simulink model "XROBO02_reference"  (R2025a)
settings: Solver=ode15s  StartTime=0  StopTime=8  MaxStep=0.002  RelTol=1e-3  AbsTol=1e-3
undefined symbols (not defined in the file): cube_l, disturbance_start, disturbance_torque_nm, F1, F2, left_target_rad, move_duration, right_target_rad, shared_payload_mass, torque_limit_scale, X, Y, Z
libraries: sm_lib x210, nesl_utility x45
(part 1 of 5)
CloseFcn:
  | try,close(h1_sm_abbYuMi_trajectory),end
  | clear h1_sm_abbYuMi_2_trajectory
  | try,close(h2_sm_abbYuMi_trajectory),end
  | clear h2_sm_abbYuMi_2_trajectory
  | try,close(h3_sm_abbYuMi_trajectory),end
  | clear h3_sm_abbYuMi_2_trajectory
  | try,close(h4_sm_abbYuMi_trajectory),end
  | clear h4_sm_abbYuMi_trajectory
  | 
  | 
  | clear simlog_sm_abbYuMi_trajectory
  | clear logsout_sm_abbYuMi_trajectory
Description:
  | Dual Arm Robot Trajectory Testing
  | Copyright 2021-2025 The MathWorks, Inc.
settings Model: Creator=smiller  LastModifiedBy=SimuVerity Contributors
settings SolverCC: AutoScaleAbsTol=off
settings DataIOCC: MaxDataPoints=10000  SignalLoggingName=logsout_sm_abbYuMi_trajectory
settings OptimizationCC: ReuseModelBlockBuffer=off
settings DebuggingCC: UnconnectedInputMsg=warning  UnconnectedOutputMsg=warning  UnconnectedLineMsg=warning
settings ModelReferenceCC: EnableRefExpFcnMdlSchedulingChecks=on
settings RTWCC: GPUComputeCapability=3.5  DLArmComputeVersion=19.05
settings SimscapeCC: SimscapeLogSimulationStatistics=on  SimscapeLogName=simlog_sm_abbYuMi_trajectory  SimscapeLogDataHistory=10000.0
settings ExplorerConfigSet: InternalSimMechanicsExplorerSettings="<ExplorerConfiguration><canonicalview>default</canonicalview><AnimationSetting><BasePlaybackSpeed>1.0</BasePlaybackSpeed><PlaybackSpeedFactor>1.0</PlaybackSpeedFactor></AnimationSetting><TilePanel><TileInfo><Tiles Columns=\"3\" Count=\"4\" Rows=\"2\"><Column Weight=\"0.6174\"/><Column Weight=\"0.1908\"/><Column Weight=\"0.1918\"/><Row Weight=\"0.4992\"/><Row Weight=\"0.5008\"/><Tile Height=\"2\" Width=\"1\" X=\"0\" Y=\"0\"/><Tile Height=\"1\" Width=\"1\" X=\"1\" Y=\"0\"/><Tile Height=\"1\" Width=\"1\" X=\"2\" Y=\"0\"/><Tile Height=\"1\" Width=\"2\" X=\"1\" Y=\"1\"/></Tiles></TileInfo><SceneInfo><SceneViewer><BGColor><R>1</R><G>1</G><B>1</B></BGColor><Camera><DoPerspective>off</DoPerspective><Position><X>1.10785151491655953</X><Y>0.401938303575801459</Y><Z>0.73930542035196356</Z></Position><Center><X>0.0422085680859981827</X><Y>-0.0186832884618209454</Y><Z>0.276020887594053299</Z></Center><Up><X>-0.346127033108781346</X><Y>-0.144162748431228449</Y><Z>0.927045402834222987</Z></Up><ViewLimDist>1</ViewLimDist><YLim>0.529480286240577747</YLim><XLim>0.750259888990338908</XLim></Camera></SceneViewer><SceneViewer><BGColor><R>1</R><G>1</G><B>1</B></BGColor><Camera><DoPerspective>off</DoPerspective><Position><X>1.28857080950961111</X><Y>0.165761602408297848</Y><Z>0.538044175913367062</Z></Position><Center><X>0.222927862679049932</X><Y>-0.254859989629324657</Y><Z>0.0747596431554567176</Z></Center><Up><X>-0.346127033108781346</X><Y>-0.144162748431228449</Y><Z>0.927045402834222987</Z></Up><ViewLimDist>1</ViewLimDist><YLim>0.0401775125475980072</YLim><XLim>0.0353441275794659157</XLim></Camera></SceneViewer><SceneViewer><BGColor><R>1</R><G>1</G><B>1</B></BGColor><Camera><DoPerspective>off</DoPerspective><Position><X>1.11107526675001367</X><Y>0.699993298566071065</Y><Z>0.461282465118678986</Z></Position><Center><X>0.045432319919452957</X><Y>0.279371706528448394</Y><Z>-0.002002067639231578</Z></Center><Up><X>-0.346127033108781346</X><Y>-0.144162748431228449</Y><Z>0.927045402834222987</Z></Up><ViewLimDist>1</ViewLimDist><YLim>0.0406072638280753281</YLim><XLim>0.0358748383443522681</XLim></Camera></SceneViewer><SceneViewer><BGColor><R>1</R><G>1</G><B>1</B></BGColor><Camera><DoPerspective>off</DoPerspective><Position><X>1.27319716760923374</X><Y>0.344894477488872697</Y><Z>0.410769600840851012</Z></Position><Center><X>0.207554220778672804</X><Y>-0.0757271145487498354</Y><Z>-0.0525149319170593112</Z></Center><Up><X>-0.346127033108781346</X><Y>-0.144162748431228449</Y><Z>0.927045402834222987</Z></Up><ViewLimDist>1</ViewLimDist><YLim>0.0389773841730341117</YLim><XLim>0.0697797364595891534</XLim></Camera></SceneViewer></SceneInfo></TilePanel><MechEditorPanel><Cameras/><GfxPanelCameraMap/><VideoCreator><PlaybackSpeedRatio>1</PlaybackSpeedRatio><FrameRate>30</FrameRate><VideoFormat>MPEG-4</VideoFormat><FrameSize>auto</FrameSize></VideoCreator></MechEditorPanel></ExplorerConfiguration>"

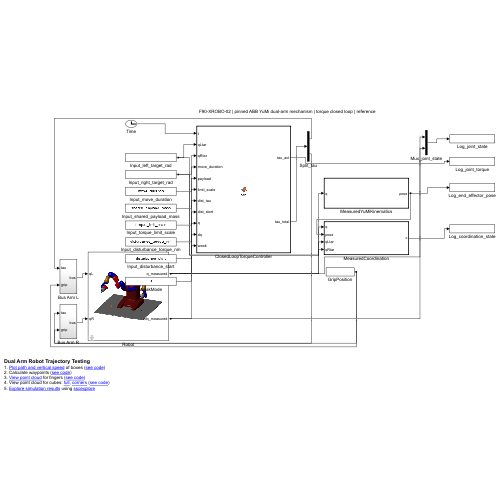
[thumbnail: Simulink's stored preview of the top-level diagram]
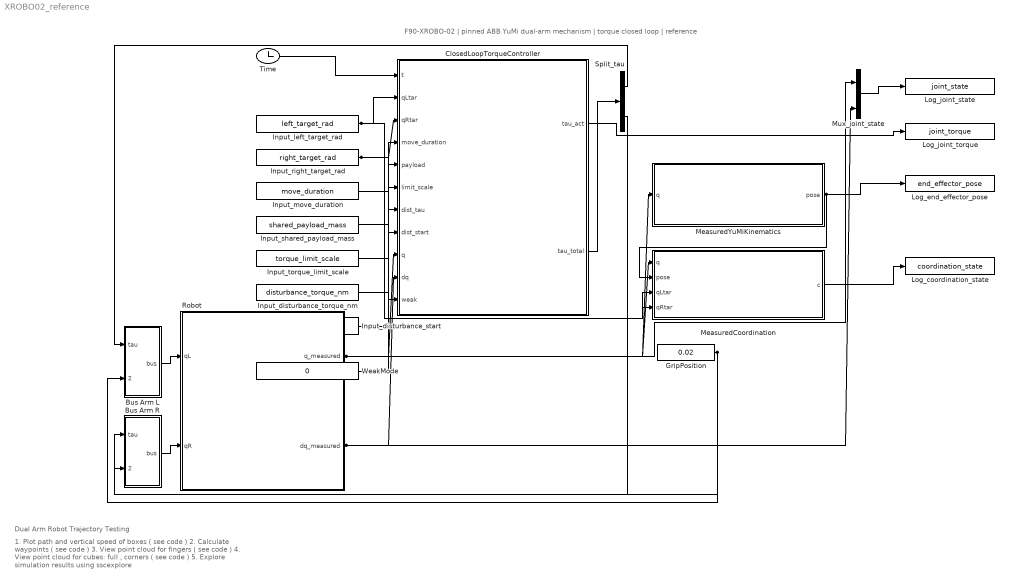
== system XROBO02_reference ==
  note: Dual Arm Robot Trajectory Testing
  note: 1. Plot path and vertical speed of boxes ( see code )
      | 2. Calculate waypoints ( see code )
      | 3. View point cloud for fingers ( see code )
      | 4. View point cloud for cubes: full , corners ( see code )
      | 5. Explore simulation results using sscexplore
  note: F90-XROBO-02 | pinned ABB YuMi dual-arm mechanism | torque closed loop | reference
  Bus Arm L : Subsystem
  Bus Arm R : Subsystem
  ClosedLoopTorqueController : MATLAB Function  TreatAsAtomicUnit=on
  GripPosition : Constant  Value=0.02
  Input_disturbance_start : Constant  Value=disturbance_start
  Input_disturbance_torque_nm : Constant  Value=disturbance_torque_nm
  Input_left_target_rad : Constant  Value=left_target_rad
  Input_move_duration : Constant  Value=move_duration
  Input_right_target_rad : Constant  Value=right_target_rad
  Input_shared_payload_mass : Constant  Value=shared_payload_mass
  Input_torque_limit_scale : Constant  Value=torque_limit_scale
  Log_coordination_state : ToWorkspace  VariableName=coordination_state  SaveFormat=Timeseries  SampleTime=-1
  Log_end_effector_pose : ToWorkspace  VariableName=end_effector_pose  SaveFormat=Timeseries  SampleTime=-1
  Log_joint_state : ToWorkspace  VariableName=joint_state  SaveFormat=Timeseries  SampleTime=-1
  Log_joint_torque : ToWorkspace  VariableName=joint_torque  SaveFormat=Timeseries  SampleTime=-1
  MeasuredCoordination : MATLAB Function  TreatAsAtomicUnit=on
  MeasuredYuMiKinematics : MATLAB Function  TreatAsAtomicUnit=on
  Mux_joint_state : Mux  Inputs=2
  Robot : Subsystem  mask(Dual Arm Robot with Contact Forces){k_gripBox=1e3, k_boxBox=1e3, k_boxFloor=1e3, d_gripBox=1e2, d_boxBox=1e2, d_boxFloor=1e2, t_gripBox=1e-3, t_boxBox=1e-3, t_boxFloor=1e-3, mu_s_gripBox=0.7, mu_s_boxBox=0.5, mu_s_boxFloor=0.5, mu_d_gripBox=0.5, mu_d_boxBox=0.3, mu_d_boxFloor=0.3, mu_v_gripBox=1e-3, mu_v_boxBox=1e-3, mu_v_boxFloor=1e-3}
      mask help: Models a dual-arm robot. Parameter values define the contact and friction forces between the gripper, boxes, and floor.
      mask DialogControl Control2_copy_copy_copy_copy_copy_copy_copy Prompt: Gripper-Box
      mask DialogControl Control2_copy_copy_copy_copy_copy_copy_copy_copy Prompt: Box-Box
      mask DialogControl Control2_copy_copy_copy_copy_copy_copy_copy_copy_copy Prompt: Box-Floor
      mask DialogControl Control2_copy_copy_copy_copy_copy_copy Prompt: Damping (N/(m/s))
      mask DialogControl Control2_copy Prompt: Damping (N/(m/s))
      mask DialogControl Control2_copy_copy Prompt: Transition Width (m)
      mask DialogControl Control2_copy_copy_copy Prompt: Static Friction (0-1)
      mask DialogControl Control2_copy_copy_copy_copy Prompt: Dynamic Friction (0-1)
      mask DialogControl Control2_copy_copy_copy_copy_copy Prompt: Critical Velocity (m/s)
      mask Display: image('sm_abbYuMi_trajectory_robot.png');
  Split_tau : Demux  Outputs=[7 7]
  Time : Clock
  WeakMode : Constant  Value=0
  wires:
  Time/1 -> ClosedLoopTorqueController/1(t)
  Input_left_target_rad/1 -> ClosedLoopTorqueController/2(qLtar), MeasuredCoordination/3(qLtar)
  Input_right_target_rad/1 -> ClosedLoopTorqueController/3(qRtar), MeasuredCoordination/4(qRtar)
  Input_move_duration/1 -> ClosedLoopTorqueController/4(move_duration)
  Input_shared_payload_mass/1 -> ClosedLoopTorqueController/5(payload)
  Input_torque_limit_scale/1 -> ClosedLoopTorqueController/6(limit_scale)
  Input_disturbance_torque_nm/1 -> ClosedLoopTorqueController/7(dist_tau)
  Input_disturbance_start/1 -> ClosedLoopTorqueController/8(dist_start)
  Robot/1(q_measured) -> ClosedLoopTorqueController/9(q), MeasuredYuMiKinematics/1(q), MeasuredCoordination/1(q), Mux_joint_state/1
  Robot/2(dq_measured) -> ClosedLoopTorqueController/10(dq), Mux_joint_state/2
  WeakMode/1 -> ClosedLoopTorqueController/11(weak)
  ClosedLoopTorqueController/2(tau_total) -> Split_tau/1
  Split_tau/1 -> Bus Arm L/1(tau)
  Split_tau/2 -> Bus Arm R/1(tau)
  GripPosition/1 -> Bus Arm L/2(grip), Bus Arm R/2(grip)
  Bus Arm L/1(bus) -> Robot/1(qL)
  Bus Arm R/1(bus) -> Robot/2(qR)
  MeasuredYuMiKinematics/1(pose) -> MeasuredCoordination/2(pose), Log_end_effector_pose/1
  Mux_joint_state/1 -> Log_joint_state/1
  ClosedLoopTorqueController/1(tau_act) -> Log_joint_torque/1
  MeasuredCoordination/1(c) -> Log_coordination_state/1

== system XROBO02_reference/Bus Arm L ==
  tau : Inport
  grip : Inport  Port=2
  Demux_tau : Demux  Outputs=7
  TorqueBus : BusCreator  Inputs=8
  bus : Outport
  wires:
  tau/1 -> Demux_tau/1
  Demux_tau/1 -> TorqueBus/1  "q1"
  Demux_tau/2 -> TorqueBus/2  "q2"
  Demux_tau/3 -> TorqueBus/3  "q3"
  Demux_tau/4 -> TorqueBus/4  "q4"
  Demux_tau/5 -> TorqueBus/5  "q5"
  Demux_tau/6 -> TorqueBus/6  "q6"
  Demux_tau/7 -> TorqueBus/7  "q7"
  grip/1 -> TorqueBus/8  "f"
  TorqueBus/1 -> bus/1

== system XROBO02_reference/Bus Arm R ==
  tau : Inport
  grip : Inport  Port=2
  Demux_tau : Demux  Outputs=7
  TorqueBus : BusCreator  Inputs=8
  bus : Outport
  wires:
  tau/1 -> Demux_tau/1
  Demux_tau/1 -> TorqueBus/1  "q1"
  Demux_tau/2 -> TorqueBus/2  "q2"
  Demux_tau/3 -> TorqueBus/3  "q3"
  Demux_tau/4 -> TorqueBus/4  "q4"
  Demux_tau/5 -> TorqueBus/5  "q5"
  Demux_tau/6 -> TorqueBus/6  "q6"
  Demux_tau/7 -> TorqueBus/7  "q7"
  grip/1 -> TorqueBus/8  "f"
  TorqueBus/1 -> bus/1

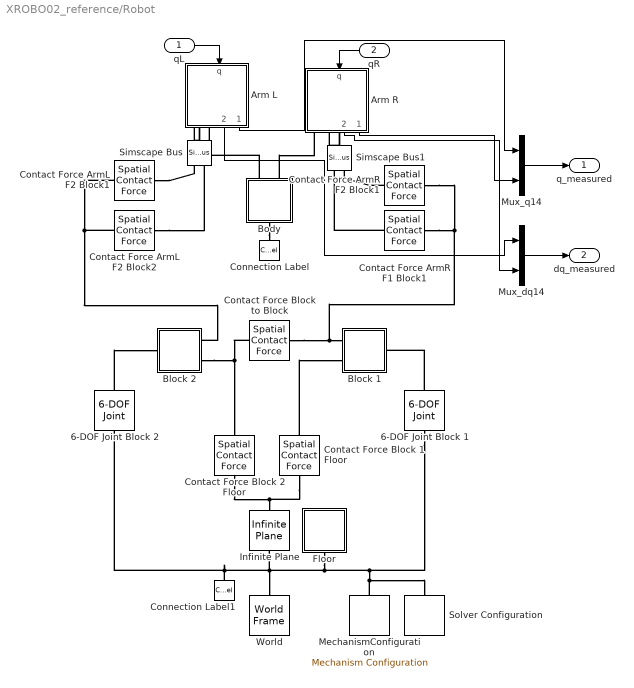
== system XROBO02_reference/Robot ==
  qL : Inport
  qR : Inport  Port=2
  " Contact Force Block to Block" : sm_lib/Forces and Torques/Spatial Contact Force  SenseSeparationDistance=off  NormalForceType=SmoothSpringDamper  NormalStiffness=k_boxBox  NormalStiffnessUnits=N/m  NormalDamping=d_boxBox  NormalDampingUnits=N/(m/s)  NormalTransitionRegionWidth=t_boxBox  NormalTransitionRegionWidthUnits=m  FrictionType=SmoothStickSlip  CoefficientOfStaticFriction=mu_s_boxBox  CoefficientOfDynamicFriction=mu_d_boxBox  FrictionalCriticalVelocity=mu_v_boxBox  FrictionalCriticalVelocityUnits=m/s  SenseContactSignal=off  SensePenetrationDepth=off  SenseNormalVelocity=off  SenseTangentialVelocity=off  SensingForceTorqueDirection=BaseOnFollower  SensingForceTorqueResolutionFrame=ContactFrame  SenseNormalForce=off  SenseNormalForceMagnitude=off  SenseNormalTorque=off  SenseFrictionalForce=off  SenseFrictionalForceMagnitude=off  SenseFrictionalTorque=off  SenseTotalForce=off  SenseTotalTorque=off  SenseContactBaseRotation=off  SenseContactBaseTranslation=off  SenseContactFollowerRotation=off  SenseContactFollowerTranslation=off  ZeroCrossDetectContactStartAndEnd=off
  6-DOF Joint Block 1 : sm_lib/Joints/6-DOF Joint  JointMode=Normal  CompositeWrenchDir=FollowerOnBase  CompositeWrenchFrame=BaseFrame  SenseConstraintForce=off  SenseConstraintTorque=off  SenseTotalForce=off  SenseTotalTorque=off  PxPositionTargetSpecify=on  PxPositionTargetPriority=High  PxPositionTargetValue=0.1  PxPositionTargetValueUnits=m  PxVelocityTargetSpecify=off  PxVelocityTargetPriority=High  PxVelocityTargetValue=0  PxVelocityTargetValueUnits=m/s  PxEquilibriumPosition=0  PxEquilibriumPositionUnits=m  PxSpringStiffness=0  PxSpringStiffnessUnits=N/m  PxDampingCoefficient=0  PxDampingCoefficientUnits=N/(m/s)  PxLowerLimitSpecify=off  PxLowerLimitBound=-1  PxLowerLimitBoundUnits=m  PxLowerLimitStiffness=1e6  PxLowerLimitStiffnessUnits=N/m  PxLowerLimitDamping=1e3  PxLowerLimitDampingUnits=N/(m/s)  PxLowerLimitTransitionRegionWidth=1e-4  PxLowerLimitTransitionRegionWidthUnits=m  PxUpperLimitSpecify=off  PxUpperLimitBound=1  PxUpperLimitBoundUnits=m  PxUpperLimitStiffness=1e6  PxUpperLimitStiffnessUnits=N/m  PxUpperLimitDamping=1e3  PxUpperLimitDampingUnits=N/(m/s)  PxUpperLimitTransitionRegionWidth=1e-4  PxUpperLimitTransitionRegionWidthUnits=m  PxTorqueActuationMode=NoTorque  PxMotionActuationMode=ComputedMotion  PxSensePosition=off  PxSenseVelocity=off  PxSenseAcceleration=off  PxSenseTorqueForce=off  PxSenseLowerLimitTorqueForce=off  PxSenseUpperLimitTorqueForce=off  PyPositionTargetSpecify=on  PyPositionTargetPriority=High  PyPositionTargetValue=-0.3  PyPositionTargetValueUnits=m  PyVelocityTargetSpecify=off  PyVelocityTargetPriority=High  PyVelocityTargetValue=0  PyVelocityTargetValueUnits=m/s  PyEquilibriumPosition=0  PyEquilibriumPositionUnits=m  PySpringStiffness=0  PySpringStiffnessUnits=N/m  PyDampingCoefficient=0  PyDampingCoefficientUnits=N/(m/s)  PyLowerLimitSpecify=off  PyLowerLimitBound=-1  PyLowerLimitBoundUnits=m  PyLowerLimitStiffness=1e6  PyLowerLimitStiffnessUnits=N/m  PyLowerLimitDamping=1e3  PyLowerLimitDampingUnits=N/(m/s)  PyLowerLimitTransitionRegionWidth=1e-4  PyLowerLimitTransitionRegionWidthUnits=m  PyUpperLimitSpecify=off  PyUpperLimitBound=1  PyUpperLimitBoundUnits=m  PyUpperLimitStiffness=1e6  PyUpperLimitStiffnessUnits=N/m  PyUpperLimitDamping=1e3  PyUpperLimitDampingUnits=N/(m/s)  PyUpperLimitTransitionRegionWidth=1e-4  PyUpperLimitTransitionRegionWidthUnits=m  PyTorqueActuationMode=NoTorque  PyMotionActuationMode=ComputedMotion  PySensePosition=off  PySenseVelocity=off  PySenseAcceleration=off  PySenseTorqueForce=off  PySenseLowerLimitTorqueForce=off  PySenseUpperLimitTorqueForce=off  PzPositionTargetSpecify=on  PzPositionTargetPriority=High  PzPositionTargetValue=0.011  PzPositionTargetValueUnits=m  PzVelocityTargetSpecify=off  PzVelocityTargetPriority=High  PzVelocityTargetValue=0  PzVelocityTargetValueUnits=m/s  PzEquilibriumPosition=0  PzEquilibriumPositionUnits=m  PzSpringStiffness=0  PzSpringStiffnessUnits=N/m  PzDampingCoefficient=0  PzDampingCoefficientUnits=N/(m/s)  PzLowerLimitSpecify=off  PzLowerLimitBound=0  PzLowerLimitBoundUnits=m  PzLowerLimitStiffness=1e6  PzLowerLimitStiffnessUnits=N/m  PzLowerLimitDamping=1e3  PzLowerLimitDampingUnits=N/(m/s)  PzLowerLimitTransitionRegionWidth=1e-4  PzLowerLimitTransitionRegionWidthUnits=m  PzUpperLimitSpecify=off  PzUpperLimitBound=1  PzUpperLimitBoundUnits=m  PzUpperLimitStiffness=1e6  PzUpperLimitStiffnessUnits=N/m  PzUpperLimitDamping=1e3  PzUpperLimitDampingUnits=N/(m/s)  PzUpperLimitTransitionRegionWidth=1e-4  PzUpperLimitTransitionRegionWidthUnits=m  PzTorqueActuationMode=NoTorque  PzMotionActuationMode=ComputedMotion  PzSensePosition=off  PzSenseVelocity=off  PzSenseAcceleration=off  PzSenseTorqueForce=off  PzSenseLowerLimitTorqueForce=off  PzSenseUpperLimitTorqueForce=off  SphPositionTargetSpecify=off  SphPositionTargetPriority=High  SphPositionTargetRotationMethod=None  SphPositionTargetFollAlignAxisA=+X  SphPositionTargetBaseAlignAxisA=+Y  SphPositionTargetFollAlignAxisB=+Y  SphPositionTargetBaseAlignAxisB=+Z  SphPositionTargetRotationStandardAxis=+Z  SphPositionTargetRotationAngle=0.0  SphPositionTargetRotationAngleUnits=deg  SphPositionTargetRotationArbitraryAxis=[0 0 1]  SphPositionTargetRotationSequenceAxes=FollowerAxes  SphPositionTargetRotationSequence=XYX  SphPositionTargetRotationSequenceAngles=[0 0 0]  SphPositionTargetRotationSequenceAnglesUnits=deg  SphPositionTargetRotationMatrix=[1 0 0; 0 1 0; 0 0 1]  SphPositionTargetQuaternion=[1 0 0 0]  SphVelocityTargetSpecify=off  SphVelocityTargetPriority=High  SphVelocityTargetValue=[0 0 0]  SphVelocityTargetValueUnits=deg/s  SphVelocityTargetInFollowerFrame=on  SphEqPosRotationMethod=None  SphEqPosFollAlignAxisA=+X  SphEqPosBaseAlignAxisA=+Y  SphEqPosFollAlignAxisB=+Y  SphEqPosBaseAlignAxisB=+Z  SphEqPosRotationStandardAxis=+Z  SphEqPosRotationAngle=0.0  SphEqPosRotationAngleUnits=deg  SphEqPosRotationArbitraryAxis=[0 0 1]  SphEqPosRotationSequenceAxes=FollowerAxes  SphEqPosRotationSequence=XYX  SphEqPosRotationSequenceAngles=[0 0 0]  SphEqPosRotationSequenceAnglesUnits=deg  SphEqPosRotationMatrix=[1 0 0; 0 1 0; 0 0 1]  SphEqPosQuaternion=[1 0 0 0]  SphSpringStiffness=0  SphSpringStiffnessUnits=N*m/deg  SphDampingCoefficient=0  SphDampingCoefficientUnits=N*m/(deg/s)  SphLowerLimitSpecify=off  SphLowerLimitBound=15  SphLowerLimitBoundUnits=deg  SphLowerLimitStiffness=1e4  SphLowerLimitStiffnessUnits=N*m/deg  SphLowerLimitDamping=10  SphLowerLimitDampingUnits=N*m/(deg/s)  SphLowerLimitTransitionRegionWidth=0.1  SphLowerLimitTransitionRegionWidthUnits=deg  SphUpperLimitSpecify=off  SphUpperLimitBound=45  SphUpperLimitBoundUnits=deg  SphUpperLimitStiffness=1e4  SphUpperLimitStiffnessUnits=N*m/deg  SphUpperLimitDamping=10  SphUpperLimitDampingUnits=N*m/(deg/s)  SphUpperLimitTransitionRegionWidth=0.1  SphUpperLimitTransitionRegionWidthUnits=deg  SphTorqueActuationMode=NoTorque  SphActuateTorqueX=off  SphActuateTorqueY=off  SphActuateTorqueZ=off  SphActuateTorque=off  SphActuationFrame=BaseFrame  SphSensePosition=off  SphSenseVelocityX=off  SphSenseVelocityY=off  SphSenseVelocityZ=off  SphSenseVelocity=off  SphSenseAccelerationX=off  SphSenseAccelerationY=off  SphSenseAccelerationZ=off  SphSenseAcceleration=off  SphSenseLowerLimitTorqueMag=off  SphSenseUpperLimitTorqueMag=off  SphSensingFrame=BaseFrame
  6-DOF Joint Block 2 : sm_lib/Joints/6-DOF Joint  JointMode=Normal  CompositeWrenchDir=FollowerOnBase  CompositeWrenchFrame=BaseFrame  SenseConstraintForce=off  SenseConstraintTorque=off  SenseTotalForce=off  SenseTotalTorque=off  PxPositionTargetSpecify=on  PxPositionTargetPriority=High  PxPositionTargetValue=0.1  PxPositionTargetValueUnits=m  PxVelocityTargetSpecify=off  PxVelocityTargetPriority=High  PxVelocityTargetValue=0  PxVelocityTargetValueUnits=m/s  PxEquilibriumPosition=0  PxEquilibriumPositionUnits=m  PxSpringStiffness=0  PxSpringStiffnessUnits=N/m  PxDampingCoefficient=0  PxDampingCoefficientUnits=N/(m/s)  PxLowerLimitSpecify=off  PxLowerLimitBound=-1  PxLowerLimitBoundUnits=m  PxLowerLimitStiffness=1e6  PxLowerLimitStiffnessUnits=N/m  PxLowerLimitDamping=1e3  PxLowerLimitDampingUnits=N/(m/s)  PxLowerLimitTransitionRegionWidth=1e-4  PxLowerLimitTransitionRegionWidthUnits=m  PxUpperLimitSpecify=off  PxUpperLimitBound=1  PxUpperLimitBoundUnits=m  PxUpperLimitStiffness=1e6  PxUpperLimitStiffnessUnits=N/m  PxUpperLimitDamping=1e3  PxUpperLimitDampingUnits=N/(m/s)  PxUpperLimitTransitionRegionWidth=1e-4  PxUpperLimitTransitionRegionWidthUnits=m  PxTorqueActuationMode=NoTorque  PxMotionActuationMode=ComputedMotion  PxSensePosition=off  PxSenseVelocity=off  PxSenseAcceleration=off  PxSenseTorqueForce=off  PxSenseLowerLimitTorqueForce=off  PxSenseUpperLimitTorqueForce=off  PyPositionTargetSpecify=on  PyPositionTargetPriority=High  PyPositionTargetValue=0.3  PyPositionTargetValueUnits=m  PyVelocityTargetSpecify=off  PyVelocityTargetPriority=High  PyVelocityTargetValue=0  PyVelocityTargetValueUnits=m/s  PyEquilibriumPosition=0  PyEquilibriumPositionUnits=m  PySpringStiffness=0  PySpringStiffnessUnits=N/m  PyDampingCoefficient=0  PyDampingCoefficientUnits=N/(m/s)  PyLowerLimitSpecify=off  PyLowerLimitBound=-1  PyLowerLimitBoundUnits=m  PyLowerLimitStiffness=1e6  PyLowerLimitStiffnessUnits=N/m  PyLowerLimitDamping=1e3  PyLowerLimitDampingUnits=N/(m/s)  PyLowerLimitTransitionRegionWidth=1e-4  PyLowerLimitTransitionRegionWidthUnits=m  PyUpperLimitSpecify=off  PyUpperLimitBound=1  PyUpperLimitBoundUnits=m  PyUpperLimitStiffness=1e6  PyUpperLimitStiffnessUnits=N/m  PyUpperLimitDamping=1e3  PyUpperLimitDampingUnits=N/(m/s)  PyUpperLimitTransitionRegionWidth=1e-4  PyUpperLimitTransitionRegionWidthUnits=m  PyTorqueActuationMode=NoTorque  PyMotionActuationMode=ComputedMotion  PySensePosition=off  PySenseVelocity=off  PySenseAcceleration=off  PySenseTorqueForce=off  PySenseLowerLimitTorqueForce=off  PySenseUpperLimitTorqueForce=off  PzPositionTargetSpecify=on  PzPositionTargetPriority=High  PzPositionTargetValue=0.011  PzPositionTargetValueUnits=m  PzVelocityTargetSpecify=off  PzVelocityTargetPriority=High  PzVelocityTargetValue=0  PzVelocityTargetValueUnits=m/s  PzEquilibriumPosition=0  PzEquilibriumPositionUnits=m  PzSpringStiffness=0  PzSpringStiffnessUnits=N/m  PzDampingCoefficient=0  PzDampingCoefficientUnits=N/(m/s)  PzLowerLimitSpecify=off  PzLowerLimitBound=0  PzLowerLimitBoundUnits=m  PzLowerLimitStiffness=1e6  PzLowerLimitStiffnessUnits=N/m  PzLowerLimitDamping=1e3  PzLowerLimitDampingUnits=N/(m/s)  PzLowerLimitTransitionRegionWidth=1e-4  PzLowerLimitTransitionRegionWidthUnits=m  PzUpperLimitSpecify=off  PzUpperLimitBound=1  PzUpperLimitBoundUnits=m  PzUpperLimitStiffness=1e6  PzUpperLimitStiffnessUnits=N/m  PzUpperLimitDamping=1e3  PzUpperLimitDampingUnits=N/(m/s)  PzUpperLimitTransitionRegionWidth=1e-4  PzUpperLimitTransitionRegionWidthUnits=m  PzTorqueActuationMode=NoTorque  PzMotionActuationMode=ComputedMotion  PzSensePosition=off  PzSenseVelocity=off  PzSenseAcceleration=off  PzSenseTorqueForce=off  PzSenseLowerLimitTorqueForce=off  PzSenseUpperLimitTorqueForce=off  SphPositionTargetSpecify=off  SphPositionTargetPriority=High  SphPositionTargetRotationMethod=None  SphPositionTargetFollAlignAxisA=+X  SphPositionTargetBaseAlignAxisA=+Y  SphPositionTargetFollAlignAxisB=+Y  SphPositionTargetBaseAlignAxisB=+Z  SphPositionTargetRotationStandardAxis=+Z  SphPositionTargetRotationAngle=0.0  SphPositionTargetRotationAngleUnits=deg  SphPositionTargetRotationArbitraryAxis=[0 0 1]  SphPositionTargetRotationSequenceAxes=FollowerAxes  SphPositionTargetRotationSequence=XYX  SphPositionTargetRotationSequenceAngles=[0 0 0]  SphPositionTargetRotationSequenceAnglesUnits=deg  SphPositionTargetRotationMatrix=[1 0 0; 0 1 0; 0 0 1]  SphPositionTargetQuaternion=[1 0 0 0]  SphVelocityTargetSpecify=off  SphVelocityTargetPriority=High  SphVelocityTargetValue=[0 0 0]  SphVelocityTargetValueUnits=deg/s  SphVelocityTargetInFollowerFrame=on  SphEqPosRotationMethod=None  SphEqPosFollAlignAxisA=+X  SphEqPosBaseAlignAxisA=+Y  SphEqPosFollAlignAxisB=+Y  SphEqPosBaseAlignAxisB=+Z  SphEqPosRotationStandardAxis=+Z  SphEqPosRotationAngle=0.0  SphEqPosRotationAngleUnits=deg  SphEqPosRotationArbitraryAxis=[0 0 1]  SphEqPosRotationSequenceAxes=FollowerAxes  SphEqPosRotationSequence=XYX  SphEqPosRotationSequenceAngles=[0 0 0]  SphEqPosRotationSequenceAnglesUnits=deg  SphEqPosRotationMatrix=[1 0 0; 0 1 0; 0 0 1]  SphEqPosQuaternion=[1 0 0 0]  SphSpringStiffness=0  SphSpringStiffnessUnits=N*m/deg  SphDampingCoefficient=0  SphDampingCoefficientUnits=N*m/(deg/s)  SphLowerLimitSpecify=off  SphLowerLimitBound=15  SphLowerLimitBoundUnits=deg  SphLowerLimitStiffness=1e4  SphLowerLimitStiffnessUnits=N*m/deg  SphLowerLimitDamping=10  SphLowerLimitDampingUnits=N*m/(deg/s)  SphLowerLimitTransitionRegionWidth=0.1  SphLowerLimitTransitionRegionWidthUnits=deg  SphUpperLimitSpecify=off  SphUpperLimitBound=45  SphUpperLimitBoundUnits=deg  SphUpperLimitStiffness=1e4  SphUpperLimitStiffnessUnits=N*m/deg  SphUpperLimitDamping=10  SphUpperLimitDampingUnits=N*m/(deg/s)  SphUpperLimitTransitionRegionWidth=0.1  SphUpperLimitTransitionRegionWidthUnits=deg  SphTorqueActuationMode=NoTorque  SphActuateTorqueX=off  SphActuateTorqueY=off  SphActuateTorqueZ=off  SphActuateTorque=off  SphActuationFrame=BaseFrame  SphSensePosition=off  SphSenseVelocityX=off  SphSenseVelocityY=off  SphSenseVelocityZ=off  SphSenseVelocity=off  SphSenseAccelerationX=off  SphSenseAccelerationY=off  SphSenseAccelerationZ=off  SphSenseAcceleration=off  SphSenseLowerLimitTorqueMag=off  SphSenseUpperLimitTorqueMag=off  SphSensingFrame=BaseFrame
  Arm L : Subsystem
  Arm R : Subsystem
  Block 1 : Subsystem
  Block 2 : Subsystem
  Body : Subsystem
  Connection Label : ConnectionLabel  Label=W
  Connection Label1 : ConnectionLabel  Label=W
  Contact Force Block 1 Floor : sm_lib/Forces and Torques/Spatial Contact Force  SenseSeparationDistance=off  NormalForceType=SmoothSpringDamper  NormalStiffness=k_boxFloor  NormalStiffnessUnits=N/m  NormalDamping=d_boxFloor  NormalDampingUnits=N/(m/s)  NormalTransitionRegionWidth=t_boxFloor  NormalTransitionRegionWidthUnits=m  FrictionType=SmoothStickSlip  CoefficientOfStaticFriction=mu_s_boxFloor  CoefficientOfDynamicFriction=mu_d_boxFloor  FrictionalCriticalVelocity=mu_v_boxFloor  FrictionalCriticalVelocityUnits=m/s  SenseContactSignal=off  SensePenetrationDepth=off  SenseNormalVelocity=off  SenseTangentialVelocity=off  SensingForceTorqueDirection=BaseOnFollower  SensingForceTorqueResolutionFrame=ContactFrame  SenseNormalForce=off  SenseNormalForceMagnitude=off  SenseNormalTorque=off  SenseFrictionalForce=off  SenseFrictionalForceMagnitude=off  SenseFrictionalTorque=off  SenseTotalForce=off  SenseTotalTorque=off  SenseContactBaseRotation=off  SenseContactBaseTranslation=off  SenseContactFollowerRotation=off  SenseContactFollowerTranslation=off  ZeroCrossDetectContactStartAndEnd=off
  Contact Force Block 2 Floor : sm_lib/Forces and Torques/Spatial Contact Force  SenseSeparationDistance=off  NormalForceType=SmoothSpringDamper  NormalStiffness=k_boxFloor  NormalStiffnessUnits=N/m  NormalDamping=d_boxFloor  NormalDampingUnits=N/(m/s)  NormalTransitionRegionWidth=t_boxFloor  NormalTransitionRegionWidthUnits=m  FrictionType=SmoothStickSlip  CoefficientOfStaticFriction=mu_s_boxFloor  CoefficientOfDynamicFriction=mu_d_boxFloor  FrictionalCriticalVelocity=mu_v_boxFloor  FrictionalCriticalVelocityUnits=m/s  SenseContactSignal=off  SensePenetrationDepth=off  SenseNormalVelocity=off  SenseTangentialVelocity=off  SensingForceTorqueDirection=BaseOnFollower  SensingForceTorqueResolutionFrame=ContactFrame  SenseNormalForce=off  SenseNormalForceMagnitude=off  SenseNormalTorque=off  SenseFrictionalForce=off  SenseFrictionalForceMagnitude=off  SenseFrictionalTorque=off  SenseTotalForce=off  SenseTotalTorque=off  SenseContactBaseRotation=off  SenseContactBaseTranslation=off  SenseContactFollowerRotation=off  SenseContactFollowerTranslation=off  ZeroCrossDetectContactStartAndEnd=off
  Contact Force ArmL F2 Block1 : sm_lib/Forces and Torques/Spatial Contact Force  SenseSeparationDistance=off  NormalForceType=SmoothSpringDamper  NormalStiffness=k_gripBox  NormalStiffnessUnits=N/m  NormalDamping=d_gripBox  NormalDampingUnits=N/(m/s)  NormalTransitionRegionWidth=t_gripBox  NormalTransitionRegionWidthUnits=m  FrictionType=SmoothStickSlip  CoefficientOfStaticFriction=mu_s_gripBox  CoefficientOfDynamicFriction=mu_d_gripBox  FrictionalCriticalVelocity=mu_v_gripBox  FrictionalCriticalVelocityUnits=m/s  SenseContactSignal=off  SensePenetrationDepth=off  SenseNormalVelocity=off  SenseTangentialVelocity=off  SensingForceTorqueDirection=BaseOnFollower  SensingForceTorqueResolutionFrame=ContactFrame  SenseNormalForce=off  SenseNormalForceMagnitude=off  SenseNormalTorque=off  SenseFrictionalForce=off  SenseFrictionalForceMagnitude=off  SenseFrictionalTorque=off  SenseTotalForce=off  SenseTotalTorque=off  SenseContactBaseRotation=off  SenseContactBaseTranslation=off  SenseContactFollowerRotation=off  SenseContactFollowerTranslation=off  ZeroCrossDetectContactStartAndEnd=off
  Contact Force ArmL F2 Block2 : sm_lib/Forces and Torques/Spatial Contact Force  SenseSeparationDistance=off  NormalForceType=SmoothSpringDamper  NormalStiffness=k_gripBox  NormalStiffnessUnits=N/m  NormalDamping=d_gripBox  NormalDampingUnits=N/(m/s)  NormalTransitionRegionWidth=t_gripBox  NormalTransitionRegionWidthUnits=m  FrictionType=SmoothStickSlip  CoefficientOfStaticFriction=mu_s_gripBox  CoefficientOfDynamicFriction=mu_d_gripBox  FrictionalCriticalVelocity=mu_v_gripBox  FrictionalCriticalVelocityUnits=m/s  SenseContactSignal=off  SensePenetrationDepth=off  SenseNormalVelocity=off  SenseTangentialVelocity=off  SensingForceTorqueDirection=BaseOnFollower  SensingForceTorqueResolutionFrame=ContactFrame  SenseNormalForce=off  SenseNormalForceMagnitude=off  SenseNormalTorque=off  SenseFrictionalForce=off  SenseFrictionalForceMagnitude=off  SenseFrictionalTorque=off  SenseTotalForce=off  SenseTotalTorque=off  SenseContactBaseRotation=off  SenseContactBaseTranslation=off  SenseContactFollowerRotation=off  SenseContactFollowerTranslation=off  ZeroCrossDetectContactStartAndEnd=off
  Contact Force ArmR F1 Block1 : sm_lib/Forces and Torques/Spatial Contact Force  SenseSeparationDistance=off  NormalForceType=SmoothSpringDamper  NormalStiffness=k_gripBox  NormalStiffnessUnits=N/m  NormalDamping=d_gripBox  NormalDampingUnits=N/(m/s)  NormalTransitionRegionWidth=t_gripBox  NormalTransitionRegionWidthUnits=m  FrictionType=SmoothStickSlip  CoefficientOfStaticFriction=mu_s_gripBox  CoefficientOfDynamicFriction=mu_d_gripBox  FrictionalCriticalVelocity=mu_v_gripBox  FrictionalCriticalVelocityUnits=m/s  SenseContactSignal=off  SensePenetrationDepth=off  SenseNormalVelocity=off  SenseTangentialVelocity=off  SensingForceTorqueDirection=BaseOnFollower  SensingForceTorqueResolutionFrame=ContactFrame  SenseNormalForce=off  SenseNormalForceMagnitude=off  SenseNormalTorque=off  SenseFrictionalForce=off  SenseFrictionalForceMagnitude=off  SenseFrictionalTorque=off  SenseTotalForce=off  SenseTotalTorque=off  SenseContactBaseRotation=off  SenseContactBaseTranslation=off  SenseContactFollowerRotation=off  SenseContactFollowerTranslation=off  ZeroCrossDetectContactStartAndEnd=off
  Contact Force ArmR F2 Block1 : sm_lib/Forces and Torques/Spatial Contact Force  SenseSeparationDistance=off  NormalForceType=SmoothSpringDamper  NormalStiffness=k_gripBox  NormalStiffnessUnits=N/m  NormalDamping=d_gripBox  NormalDampingUnits=N/(m/s)  NormalTransitionRegionWidth=t_gripBox  NormalTransitionRegionWidthUnits=m  FrictionType=SmoothStickSlip  CoefficientOfStaticFriction=mu_s_gripBox  CoefficientOfDynamicFriction=mu_d_gripBox  FrictionalCriticalVelocity=mu_v_gripBox  FrictionalCriticalVelocityUnits=m/s  SenseContactSignal=off  SensePenetrationDepth=off  SenseNormalVelocity=off  SenseTangentialVelocity=off  SensingForceTorqueDirection=BaseOnFollower  SensingForceTorqueResolutionFrame=ContactFrame  SenseNormalForce=off  SenseNormalForceMagnitude=off  SenseNormalTorque=off  SenseFrictionalForce=off  SenseFrictionalForceMagnitude=off  SenseFrictionalTorque=off  SenseTotalForce=off  SenseTotalTorque=off  SenseContactBaseRotation=off  SenseContactBaseTranslation=off  SenseContactFollowerRotation=off  SenseContactFollowerTranslation=off  ZeroCrossDetectContactStartAndEnd=off
  Floor : Subsystem
  Infinite Plane : sm_lib/Curves and Surfaces/Infinite Plane  GraphicType=Rectangle  GraphicPlaneWidth=1  GraphicPlaneWidthUnits=m  GraphicPlaneHeight=1  GraphicPlaneHeightUnits=m  GraphicVisPropType=SimpleVisualProperties  GraphicDiffuseColor=[0.5 0.5 0.5]  GraphicOpacity=0.25  GraphicSpecularColor=[0.5 0.5 0.5 1.0]  GraphicAmbientColor=[0.15 0.15 0.15 1.0]  GraphicEmissiveColor=[0.0 0.0 0.0 1.0]  GraphicShininess=75
  MechanismConfiguration : sm_lib/Utilities/Mechanism Configuration  UniformGravity=Constant  GravityVector=[0 0 -9.80665]  GravityVectorUnits=m/s^2  LinearizationDelta=0.001  JointModeTransitionNonlinearIterations=2
  Mux_dq14 : Mux  Inputs=2
  Mux_q14 : Mux  Inputs=2
  Simscape Bus : SimscapeBus  HierarchyStrings=F1;F2
  Simscape Bus1 : SimscapeBus  HierarchyStrings=F1;F2
  Solver Configuration : nesl_utility/Solver Configuration  PhysicalDomain=network_engine_domain  SubClassName=solver  LeftPortType=input  RightPortType=generic  Tones=[]  Harmonics=[]  SimulateNoise=off  Profile=off  UseLocalSampling=off  EnableSwitchedLinearOptims=on  FrequencyDomain=off  UseCCode=off  RelTol=0.001  AbsTol=1e-06  MinStep=1e-09  ToWorkspace=off  RevertToSquareIcSolve=off  NumHomotopyIterations=100  PhasorMode=off  PhasorModeNumHarmonics=1  ConsistencySolver=NEWTON_FTOL  IndexReductionMethod=DerivativeReplacement  DoDC=off  ResidualTolerance=1e-09  ConsistencyTolSource=GLOBAL  ConsistencyAbsTol=0.001  ConsistencyRelTol=0.001  ConsistencyTolFactor=0.001  UseLocalSolver=off  LocalSolverChoice=NE_BACKWARD_EULER_ADVANCER  ResolveIndetEquations=on  FunctionEvalNumThread=1  LocalSolverSampleTime=0.001  DoFixedCost=off  MaxNonlinIter=3  MaxModeIter=2  ComputeImpulses=off  ImpulseIterations=2  LinearAlgebra=auto  LinearAlgebraNumThread=0  EquationFormulation=NE_TIME_EF  DelaysMemoryBudget=1024  AutomaticFiltering=on  FilteringTimeConstant=0.001  PartitionStorageMethod=AS_NEEDED  PartitionMemoryBudget=1024  PartitionMethod=ROBUST  MultibodyUseLocalSolver=off  MultibodyLocalSolverChoice=ODE1  MultibodyLocalSolverSampleTime=0.001
  World : sm_lib/Frames and Transforms/World Frame
  q_measured : Outport
  dq_measured : Outport  Port=2
  wires:
  qR/1 -> Arm R/1(q)
  qL/1 -> Arm L/1(q)
  Arm L/1(q_measured) -> Mux_q14/1
  Arm R/1(q_measured) -> Mux_q14/2
  Arm L/2(dq_measured) -> Mux_dq14/1
  Arm R/2(dq_measured) -> Mux_dq14/2
  Mux_q14/1 -> q_measured/1
  Mux_dq14/1 -> dq_measured/1
  connections:
  6-DOF Joint Block 1/RConn1 -- Block 1/RConn1
  Contact Force ArmL F2 Block1/RConn1 -- Contact Force ArmL F2 Block2/RConn1 -- Block 2/LConn1
  Block 2/LConn2 -- " Contact Force Block to Block"/LConn1 -- Contact Force Block 2 Floor/LConn1
  MechanismConfiguration/RConn1 -- Infinite Plane/LConn1 -- World/RConn1 -- 6-DOF Joint Block 2/LConn1 -- Connection Label1/LConn1 -- Floor/LConn1 -- 6-DOF Joint Block 1/LConn1 -- Solver Configuration/RConn1
  Contact Force ArmR F2 Block1/LConn1 -- Simscape Bus1/LConn2
  Contact Force ArmL F2 Block1/LConn1 -- Simscape Bus/LConn1
  Contact Force ArmR F2 Block1/RConn1 -- " Contact Force Block to Block"/RConn1 -- Block 1/LConn1 -- Contact Force ArmR F1 Block1/RConn1
  Simscape Bus/RConn1 -- Arm L/RConn2
  Contact Force Block 2 Floor/RConn1 -- Contact Force Block 1 Floor/RConn1 -- Infinite Plane/RConn1
  Contact Force Block 1 Floor/LConn1 -- Block 1/LConn2
  Simscape Bus1/RConn1 -- Arm R/RConn1
  Contact Force ArmR F1 Block1/LConn1 -- Simscape Bus1/LConn1
  6-DOF Joint Block 2/RConn1 -- Block 2/RConn1
  Contact Force ArmL F2 Block2/LConn1 -- Simscape Bus/LConn2
  Body/RConn1 -- Arm L/RConn1
  Body/RConn2 -- Arm R/RConn2
  Body/LConn1 -- Connection Label/LConn1
